simulink model "Control_LIM_H9"  (R2025b)
settings: Solver=VariableStepAuto  StartTime=0.0  StopTime=10  RelTol=1e-3
undefined symbols (not defined in the file): a, airgap, b, corriente, dent_lsm, force_lsm, frecuencia_acel, frecuencia_freno, fuerza, fuerza_drag, FuerzaX_freno, kd, magnitude, masa_pod, paso_polar, r, slip, vel_motor_freno, velocidad_drag
libraries: slpidlib x3, eeTransforms x1
(part 1 of 2)
settings Model: NumberOfSteps=1500000  Creator=Siulesoj5  LastModifiedBy=Lenovo
settings RTWCC: GPUComputeCapability=3.5

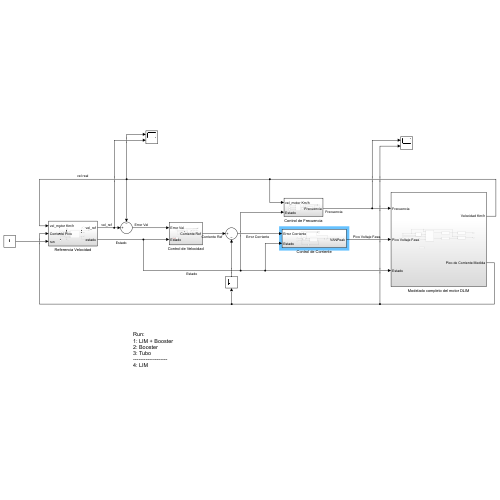
[thumbnail: Simulink's stored preview of the top-level diagram]
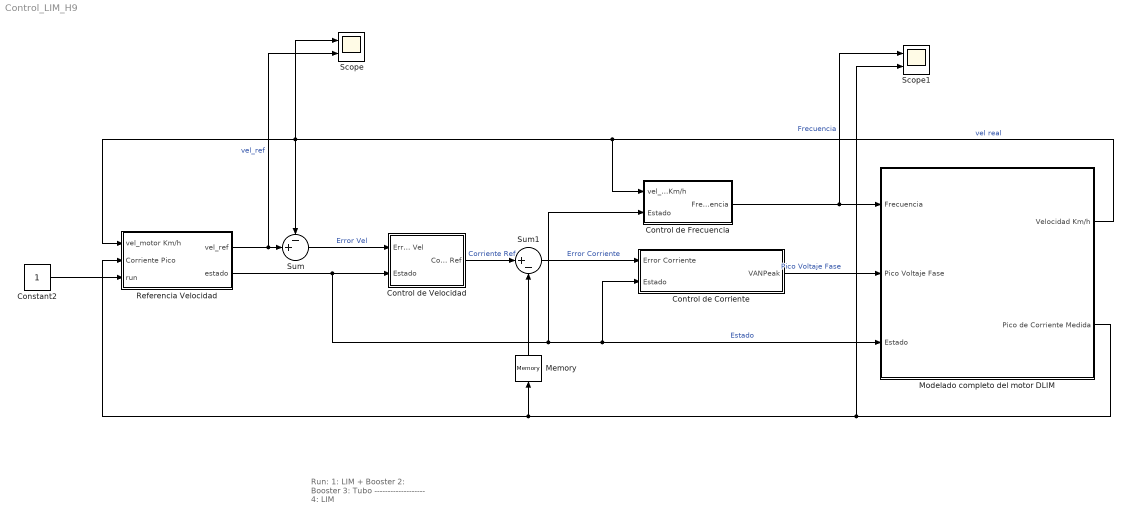
== system Control_LIM_H9 ==
  note: Run:
      | 1: LIM + Booster
      | 2: Booster
      | 3: Tubo
      | -------------------
      | 4: LIM
  Constant2 : Constant  OutMin=1  OutMax=4  OutDataTypeStr=int16
  Control de Corriente : Subsystem
  Control de Frecuencia : Subsystem
  Control de Velocidad : Subsystem
  Memory : Memory
  Modelado completo del motor DLIM : Subsystem
  Referencia Velocidad : Subsystem
  Scope : Scope  NumInputPorts=2
      settings: ActiveDisplayYMinimum=-1  ActiveDisplayYMaximum=1  DataLoggingVariableName=ScopeData19
  Scope1 : Scope  NumInputPorts=2
      settings: ActiveDisplayYMinimum=-1  ActiveDisplayYMaximum=1  DataLoggingVariableName=ScopeData20
  Sum : Sum  Inputs=-+|
  Sum1 : Sum  Inputs=|+-
  wires:
  Referencia Velocidad/1(vel_ref) -> Scope/2, Sum/2  "vel_ref"
  Sum/1 -> Control de Velocidad/1(Error Vel)  "Error Vel"
  Control de Velocidad/1(Corriente Ref) -> Sum1/1  "Corriente Ref"
  Sum1/1 -> Control de Corriente/1(Error Corriente)  "Error Corriente"
  Referencia Velocidad/2(estado) -> Modelado completo del motor DLIM/3(Estado), Control de Corriente/2(Estado), Control de Frecuencia/2(Estado), Control de Velocidad/2(Estado)  "Estado"
  Memory/1 -> Sum1/2
  Constant2/1 -> Referencia Velocidad/3(run)
  Modelado completo del motor DLIM/2(Pico de Corriente Medida) -> Referencia Velocidad/2(Corriente Pico), Memory/1, Scope1/2
  Modelado completo del motor DLIM/1(Velocidad Km/h) -> Scope/1, Sum/1, Referencia Velocidad/1(vel_motor Km/h), Control de Frecuencia/1(vel_motor Km/h)  "vel real"
  Control de Frecuencia/1(Frecuencia) -> Scope1/1, Modelado completo del motor DLIM/1(Frecuencia)  "Frecuencia"
  Control de Corriente/1(VANPeak) -> Modelado completo del motor DLIM/2(Pico Voltaje Fase)  "Pico Voltaje Fase"

== system Control_LIM_H9/Control de Corriente ==
  Error Corriente : Inport
  Estado : Inport  Port=2
  MATLAB Function : MATLAB Function  TreatAsAtomicUnit=on
  Memory : Memory
  PID Controller : slpidlib/PID Controller  Controller=PI  Form=Parallel  TimeDomain=Discrete-time  UseExternalTs=off  SampleTime=0.0002  IntegratorMethod=Forward Euler  FilterMethod=Forward Euler  ControllerParametersSource=internal  P=1  I=12  UseKiTs=off  D=0  UseExternalDerivativeSource=off  N=100  UseFilter=on  TunerSelectOption=Transfer Function Based (PID Tuner App)  InitialConditionSource=internal  InitialConditionForIntegrator=0  InitialConditionForFilter=0  DifferentiatorICPrevScaledInput=0  ExternalReset=level  TrackingMode=off  Kt=1  LimitOutput=off  SatLimitsSource=internal  UpperSaturationLimit=inf  LowerSaturationLimit=-inf  LinearizeAsGain=on  AntiWindupMode=none  Kb=1  LimitIntegrator=off  UpperIntegratorSaturationLimit=inf  LowerIntegratorSaturationLimit=-inf  POutMin=[]  POutMax=[]  IOutMin=[]  IOutMax=[]  DOutMin=[]  DOutMax=[]  NOutMin=[]  NOutMax=[]  SumOutMin=[]  SumOutMax=[]  SaturationOutMin=[]  SaturationOutMax=[]  PParamMin=[]  PParamMax=[]  IParamMin=[]  IParamMax=[]  DParamMin=[]  DParamMax=[]  NParamMin=[]  NParamMax=[]  KbParamMin=[]  KbParamMax=[]  KtParamMin=[]  KtParamMax=[]  KbOutMin=[]  KbOutMax=[]  KtOutMin=[]  KtOutMax=[]  IntegratorOutMin=[]  IntegratorOutMax=[]  FilterOutMin=[]  FilterOutMax=[]  SumI1OutMin=[]  SumI1OutMax=[]  SumI2OutMin=[]  SumI2OutMax=[]  SumI3OutMin=[]  SumI3OutMax=[]  SumI4OutMin=[]  SumI4OutMax=[]  SumDOutMin=[]  SumDOutMax=[]  DifferentiatorOutMin=[]  DifferentiatorOutMax=[]  FilterDiffOutCoefMin=[]  FilterDiffOutCoefMax=[]  ReciprocalOutMin=[]  ReciprocalOutMax=[]  SumDenOutMin=[]  SumDenOutMax=[]  SumNumOutMin=[]  SumNumOutMax=[]  DivideOutMin=[]  DivideOutMax=[]  UdiffTsProdOutMin=[]  UdiffTsProdOutMax=[]  NTsProdOutMin=[]  NTsProdOutMax=[]  UintegralTsProdOutMin=[]  UintegralTsProdOutMax=[]  UngainTsProdOutMin=[]  UngainTsProdOutMax=[]  ClampingZeroOutDataTypeStr=Inherit: Inherit via back propagation  ClampingZeroOutMin=[]  ClampingZeroOutMax=[]  FilterDenConstantOutDataTypeStr=Inherit: Inherit via back propagation  FilterDenConstantOutMin=[]  FilterDenConstantOutMax=[]  PCopyOutDataTypeStr=Inherit: Inherit via back propagation  PCopyOutMin=[]  PCopyOutMax=[]  NCopyOutDataTypeStr=Inherit: Inherit via back propagation  NCopyOutMin=[]  NCopyOutMax=[]  IntegratorContinuousStateAttributes=''  IntegratorStateMustResolveToSignalObject=off  IntegratorRTWStateStorageClass=Auto  FilterContinuousStateAttributes=''  FilterStateMustResolveToSignalObject=off  FilterRTWStateStorageClass=Auto  ParallelPVariant=InternalParameters  IdealPVariant=Disabled  IVariant=InternalParameters  DVariant=Disabled  IntegratorVariant=Discrete  SatVariant=Disabled  AWVariant=Passthrough  PCopyVariant=Disabled  TRVariant=Disabled  FdbkBlocksVariant=Forward  IdealPFdbkVariant=Disabled  SatFdbkVariant=Disabled  DerivativeFilterVariant=Disabled  NVariant=Disabled  NCopyVariant=Disabled_SignalSpec  FilterICVariant=Disabled  IntegratorICVariant=InternalICs  ExternalResetVariant=ExternalReset  TRSumVariant=Passthrough  SumFdbkVariant=Disabled  SumVariant=Sum_PI  TsampFilterVariant=InternalTs  TsampNgainVariant=Passthrough  TsampIntegralVariant=Disabled_SignalSpec  ExternalSaturationOutDataTypeStr=Inherit: Same as second input  DerivativeSourceVariant=Disabled  PreIntVariant=InternalPreInt
  Saturation : Saturate  UpperLimit=250*(sqrt(3)/2)/sqrt(3)  LowerLimit=0
  Scope : Scope  NumInputPorts=3
      settings: ActiveDisplayYMinimum=-76.56634  ActiveDisplayYMaximum=118.49234  DataLoggingVariableName=ScopeData5
  VANPeak : Outport
  wires:
  Error Corriente/1 -> Scope/1, PID Controller/1
  PID Controller/1 -> Scope/2, MATLAB Function/1(corriente)
  Saturation/1 -> Scope/3, VANPeak/1
  MATLAB Function/1(pico_voltaje) -> Saturation/1
  Estado/1 -> MATLAB Function/2(estado)
  MATLAB Function/2(reset) -> Memory/1
  Memory/1 -> PID Controller/2

== system Control_LIM_H9/Control de Frecuencia ==
  vel_motor Km/h : Inport
  Estado : Inport  Port=2
  Constant : Constant  Value=a
  Constant1 : Constant  Value=b
  Constant2 : Constant  Value=-3
  MATLAB Function : MATLAB Function  TreatAsAtomicUnit=on
  MATLAB Function1 : MATLAB Function  TreatAsAtomicUnit=on
  Scope : Scope  NumInputPorts=3
      settings: ActiveDisplayYMinimum=29.835238215543111  ActiveDisplayYMaximum=30.084237893487973
  Frecuencia : Outport
  wires:
  vel_motor Km/h/1 -> MATLAB Function/1(vel)
  MATLAB Function/1(frecuencia) -> Scope/1, MATLAB Function1/1(f_acel)  "f_aceleracion"
  MATLAB Function1/1(f) -> Scope/3, Frecuencia/1  "f_actual"
  Constant/1 -> MATLAB Function/2(a)
  Constant1/1 -> MATLAB Function/3(b)
  Constant2/1 -> Scope/2, MATLAB Function1/2(f_frenado)  "f_frenado"
  Estado/1 -> MATLAB Function1/3(estado)

== system Control_LIM_H9/Control de Velocidad ==
  Error Vel : Inport
  Estado : Inport  Port=2
  Abs : Abs  ZeroCross=off  SaturateOnIntegerOverflow=off
  Abs1 : Abs  SaturateOnIntegerOverflow=off
  MATLAB Function : MATLAB Function  TreatAsAtomicUnit=on
  MATLAB Function1 : MATLAB Function  TreatAsAtomicUnit=on
  Memory : Memory
  PID Controller : slpidlib/PID Controller  Controller=PI  Form=Parallel  TimeDomain=Discrete-time  UseExternalTs=off  SampleTime=0.001  IntegratorMethod=Forward Euler  FilterMethod=Forward Euler  ControllerParametersSource=internal  P=9  I=1  UseKiTs=off  D=0  UseExternalDerivativeSource=off  N=100  UseFilter=on  TunerSelectOption=Transfer Function Based (PID Tuner App)  InitialConditionSource=internal  InitialConditionForIntegrator=0  InitialConditionForFilter=0  DifferentiatorICPrevScaledInput=0  ExternalReset=level  TrackingMode=off  Kt=1  LimitOutput=off  SatLimitsSource=internal  UpperSaturationLimit=inf  LowerSaturationLimit=-inf  LinearizeAsGain=on  AntiWindupMode=none  Kb=1  LimitIntegrator=off  UpperIntegratorSaturationLimit=inf  LowerIntegratorSaturationLimit=-inf  POutMin=[]  POutMax=[]  IOutMin=[]  IOutMax=[]  DOutMin=[]  DOutMax=[]  NOutMin=[]  NOutMax=[]  SumOutMin=[]  SumOutMax=[]  SaturationOutMin=[]  SaturationOutMax=[]  PParamMin=[]  PParamMax=[]  IParamMin=[]  IParamMax=[]  DParamMin=[]  DParamMax=[]  NParamMin=[]  NParamMax=[]  KbParamMin=[]  KbParamMax=[]  KtParamMin=[]  KtParamMax=[]  KbOutMin=[]  KbOutMax=[]  KtOutMin=[]  KtOutMax=[]  IntegratorOutMin=[]  IntegratorOutMax=[]  FilterOutMin=[]  FilterOutMax=[]  SumI1OutMin=[]  SumI1OutMax=[]  SumI2OutMin=[]  SumI2OutMax=[]  SumI3OutMin=[]  SumI3OutMax=[]  SumI4OutMin=[]  SumI4OutMax=[]  SumDOutMin=[]  SumDOutMax=[]  DifferentiatorOutMin=[]  DifferentiatorOutMax=[]  FilterDiffOutCoefMin=[]  FilterDiffOutCoefMax=[]  ReciprocalOutMin=[]  ReciprocalOutMax=[]  SumDenOutMin=[]  SumDenOutMax=[]  SumNumOutMin=[]  SumNumOutMax=[]  DivideOutMin=[]  DivideOutMax=[]  UdiffTsProdOutMin=[]  UdiffTsProdOutMax=[]  NTsProdOutMin=[]  NTsProdOutMax=[]  UintegralTsProdOutMin=[]  UintegralTsProdOutMax=[]  UngainTsProdOutMin=[]  UngainTsProdOutMax=[]  ClampingZeroOutDataTypeStr=Inherit: Inherit via back propagation  ClampingZeroOutMin=[]  ClampingZeroOutMax=[]  FilterDenConstantOutDataTypeStr=Inherit: Inherit via back propagation  FilterDenConstantOutMin=[]  FilterDenConstantOutMax=[]  PCopyOutDataTypeStr=Inherit: Inherit via back propagation  PCopyOutMin=[]  PCopyOutMax=[]  NCopyOutDataTypeStr=Inherit: Inherit via back propagation  NCopyOutMin=[]  NCopyOutMax=[]  IntegratorContinuousStateAttributes=''  IntegratorStateMustResolveToSignalObject=off  IntegratorRTWStateStorageClass=Auto  FilterContinuousStateAttributes=''  FilterStateMustResolveToSignalObject=off  FilterRTWStateStorageClass=Auto  ParallelPVariant=InternalParameters  IdealPVariant=Disabled  IVariant=InternalParameters  DVariant=Disabled  IntegratorVariant=Discrete  SatVariant=Disabled  AWVariant=Passthrough  PCopyVariant=Disabled  TRVariant=Disabled  FdbkBlocksVariant=Forward  IdealPFdbkVariant=Disabled  SatFdbkVariant=Disabled  DerivativeFilterVariant=Disabled  NVariant=Disabled  NCopyVariant=Disabled_SignalSpec  FilterICVariant=Disabled  IntegratorICVariant=InternalICs  ExternalResetVariant=ExternalReset  TRSumVariant=Passthrough  SumFdbkVariant=Disabled  SumVariant=Sum_PI  TsampFilterVariant=InternalTs  TsampNgainVariant=Passthrough  TsampIntegralVariant=Disabled_SignalSpec  ExternalSaturationOutDataTypeStr=Inherit: Same as second input  DerivativeSourceVariant=Disabled  PreIntVariant=InternalPreInt
  PID Controller1 : slpidlib/PID Controller  Controller=PI  Form=Parallel  TimeDomain=Continuous-time  UseExternalTs=off  SampleTime=-1  IntegratorMethod=Forward Euler  FilterMethod=Forward Euler  ControllerParametersSource=internal  P=1  I=1  UseKiTs=off  D=0  UseExternalDerivativeSource=off  N=100  UseFilter=on  TunerSelectOption=Transfer Function Based (PID Tuner App)  InitialConditionSource=internal  InitialConditionForIntegrator=0  InitialConditionForFilter=0  DifferentiatorICPrevScaledInput=0  ExternalReset=none  TrackingMode=off  Kt=1  LimitOutput=off  SatLimitsSource=internal  UpperSaturationLimit=inf  LowerSaturationLimit=-inf  LinearizeAsGain=on  AntiWindupMode=none  Kb=1  LimitIntegrator=off  UpperIntegratorSaturationLimit=inf  LowerIntegratorSaturationLimit=-inf  POutMin=[]  POutMax=[]  IOutMin=[]  IOutMax=[]  DOutMin=[]  DOutMax=[]  NOutMin=[]  NOutMax=[]  SumOutMin=[]  SumOutMax=[]  SaturationOutMin=[]  SaturationOutMax=[]  PParamMin=[]  PParamMax=[]  IParamMin=[]  IParamMax=[]  DParamMin=[]  DParamMax=[]  NParamMin=[]  NParamMax=[]  KbParamMin=[]  KbParamMax=[]  KtParamMin=[]  KtParamMax=[]  KbOutMin=[]  KbOutMax=[]  KtOutMin=[]  KtOutMax=[]  IntegratorOutMin=[]  IntegratorOutMax=[]  FilterOutMin=[]  FilterOutMax=[]  SumI1OutMin=[]  SumI1OutMax=[]  SumI2OutMin=[]  SumI2OutMax=[]  SumI3OutMin=[]  SumI3OutMax=[]  SumI4OutMin=[]  SumI4OutMax=[]  SumDOutMin=[]  SumDOutMax=[]  DifferentiatorOutMin=[]  DifferentiatorOutMax=[]  FilterDiffOutCoefMin=[]  FilterDiffOutCoefMax=[]  ReciprocalOutMin=[]  ReciprocalOutMax=[]  SumDenOutMin=[]  SumDenOutMax=[]  SumNumOutMin=[]  SumNumOutMax=[]  DivideOutMin=[]  DivideOutMax=[]  UdiffTsProdOutMin=[]  UdiffTsProdOutMax=[]  NTsProdOutMin=[]  NTsProdOutMax=[]  UintegralTsProdOutMin=[]  UintegralTsProdOutMax=[]  UngainTsProdOutMin=[]  UngainTsProdOutMax=[]  ClampingZeroOutDataTypeStr=Inherit: Inherit via back propagation  ClampingZeroOutMin=[]  ClampingZeroOutMax=[]  FilterDenConstantOutDataTypeStr=Inherit: Inherit via back propagation  FilterDenConstantOutMin=[]  FilterDenConstantOutMax=[]  PCopyOutDataTypeStr=Inherit: Inherit via back propagation  PCopyOutMin=[]  PCopyOutMax=[]  NCopyOutDataTypeStr=Inherit: Inherit via back propagation  NCopyOutMin=[]  NCopyOutMax=[]  IntegratorContinuousStateAttributes=''  IntegratorStateMustResolveToSignalObject=off  IntegratorRTWStateStorageClass=Auto  FilterContinuousStateAttributes=''  FilterStateMustResolveToSignalObject=off  FilterRTWStateStorageClass=Auto  ParallelPVariant=InternalParameters  IdealPVariant=Disabled  IVariant=InternalParameters  DVariant=Disabled  IntegratorVariant=Continuous  SatVariant=Disabled  AWVariant=Passthrough  PCopyVariant=Disabled  TRVariant=Disabled  FdbkBlocksVariant=Forward  IdealPFdbkVariant=Disabled  SatFdbkVariant=Disabled  DerivativeFilterVariant=Disabled  NVariant=Disabled  NCopyVariant=Disabled_SignalSpec  FilterICVariant=Disabled  IntegratorICVariant=InternalICs  ExternalResetVariant=Disabled  TRSumVariant=Passthrough  SumFdbkVariant=Disabled  SumVariant=Sum_PI  TsampFilterVariant=InternalTs  TsampNgainVariant=Passthrough  TsampIntegralVariant=Disabled_SignalSpec  ExternalSaturationOutDataTypeStr=Inherit: Same as second input  DerivativeSourceVariant=Disabled  PreIntVariant=InternalPreInt
  Saturation : Saturate  UpperLimit=100  LowerLimit=-100
  Scope : Scope  NumInputPorts=5
      settings: ActiveDisplayYMinimum=-64.17635  ActiveDisplayYMaximum=47.1097  DataLoggingVariableName=ScopeData4
  Scope1 : Scope
      settings: ActiveDisplayYMinimum=-0.875  ActiveDisplayYMaximum=7.875  DataLoggingVariableName=ScopeData5
  Scope2 : Scope  NumInputPorts=2
      settings: ActiveDisplayYMinimum=-56.2709708249014  ActiveDisplayYMaximum=506.43873742411267  DataLoggingVariableName=ScopeData24
  Corriente Ref : Outport
  wires:
  Estado/1 -> Scope1/1, MATLAB Function/2(estado)
  MATLAB Function/1(i_ref) -> Scope2/2, Saturation/1  "i_ref sin saturar"
  Abs/1 -> Corriente Ref/1, Scope/5
  MATLAB Function/2(reset) -> Memory/1
  Memory/1 -> PID Controller/2
  Saturation/1 -> Scope2/1, Abs/1, Scope/4  "i_ref saturada"
  PID Controller/1 -> Scope/3, MATLAB Function/1(i)
  ? -> MATLAB Function1/2(normal)
  Abs1/1 -> MATLAB Function1/1(abs)
  ? -> MATLAB Function1/3(estado)
  ? -> Abs1/1
  Error Vel/1 -> Scope/1, Scope/2, PID Controller/1

== system Control_LIM_H9/Modelado completo del motor DLIM ==
  Frecuencia : Inport
  Pico Voltaje Fase : Inport  Port=2
  Estado : Inport  Port=3
  Constant1 : Constant  OutMin=1  OutMax=4  OutDataTypeStr=double
  Cálculo Máximo : Subsystem
  Cálculo Velocidad : Subsystem
  Integración Booster : Subsystem  Commented=on
  Inversor Trifásico : Subsystem
  LIM Model : Subsystem
  Sensor IMU : Subsystem
  Sensor de Corriente : Subsystem
  Velocidad Km/h : Outport
  Pico de Corriente Medida : Outport  Port=2
  wires:
  Sensor IMU/1(Acel_IMU) -> Cálculo Velocidad/1(acel m/s^2)  "Aceleración m/s^2"
  LIM Model/2(Corriente UVW) -> Sensor de Corriente/1(Corriente UVW)  "Corriente Real"
  Inversor Trifásico/1(VFaseN) -> LIM Model/2(VFaseN)
  Pico Voltaje Fase/1 -> Inversor Trifásico/2(VUNPeak)
  Constant1/1 -> LIM Model/4(Fuerza_lsm)
  Sensor de Corriente/1(Corriente Medida) -> Cálculo Máximo/2(Corriente Medida)  "Corriente Medida"
  Frecuencia/1 -> LIM Model/1(Frecuencia), Cálculo Máximo/1(Frecuencia), Inversor Trifásico/1(Frecuencia)
  LIM Model/1(Acel (m/s^2)) -> Sensor IMU/1(Acel)  "Aceleración Real"
  Cálculo Máximo/1(Corriente Pico) -> Pico de Corriente Medida/1  "Pico de Corriente Medida"
  Estado/1 -> LIM Model/3(Estado)
  Cálculo Velocidad/1(vel_motor Km/h) -> Velocidad Km/h/1  "Velocidad Km/h"

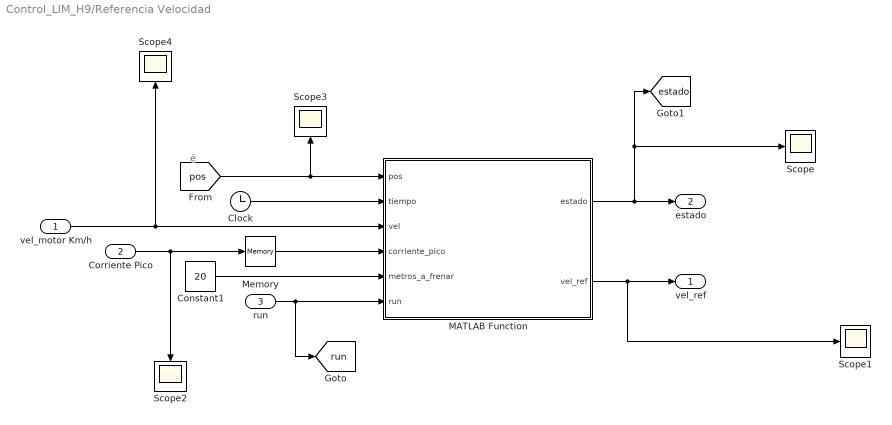
== system Control_LIM_H9/Referencia Velocidad ==
  note: é
  vel_motor Km/h : Inport
  Corriente Pico : Inport  Port=2
  run : Inport  Port=3
  Clock : Clock
  Constant1 : Constant  Value=20
  MATLAB Function : MATLAB Function  TreatAsAtomicUnit=on
  Memory : Memory
  Scope{,1..4} (5 alike) : Scope
      Scope settings: ActiveDisplayYMinimum=-0.875  ActiveDisplayYMaximum=7.875  DataLoggingVariableName=ScopeData2
      Scope1 settings: ActiveDisplayYMinimum=-6.25  ActiveDisplayYMaximum=56.25  DataLoggingVariableName=ScopeData3
      Scope2 settings: ActiveDisplayYMinimum=-11.77656  ActiveDisplayYMaximum=109.65201  DataLoggingVariableName=ScopeData11
      Scope3 settings: ActiveDisplayYMinimum=-4.42643  ActiveDisplayYMaximum=39.83783  DataLoggingVariableName=ScopeData12
      Scope4 settings: ActiveDisplayYMinimum=-6.27724  ActiveDisplayYMaximum=56.25913  DataLoggingVariableName=ScopeData4
  vel_ref : Outport
  estado : Outport  Port=2
  tag scope: estado=global, run=global
  wires:
  MATLAB Function/1(estado) -> [estado], Scope/1, estado/1
  Corriente Pico/1 -> Memory/1, Scope2/1
  Memory/1 -> MATLAB Function/4(corriente_pico)
  Constant1/1 -> MATLAB Function/5(metros_a_frenar)
  vel_motor Km/h/1 -> Scope4/1, MATLAB Function/3(vel)
  MATLAB Function/2(vel_ref) -> vel_ref/1, Scope1/1
  Clock/1 -> MATLAB Function/2(tiempo)
  [pos] -> MATLAB Function/1(pos), Scope3/1
  run/1 -> MATLAB Function/6(run), [run]

== system Control_LIM_H9/Modelado completo del motor DLIM/Cálculo Máximo ==
  Frecuencia : Inport
  Corriente Medida : Inport  Port=2
  Clock : Clock
  MATLAB Function : MATLAB Function  TreatAsAtomicUnit=on
  Scope : Scope  NumInputPorts=2
      settings: ActiveDisplayYMinimum=-131.22711  ActiveDisplayYMaximum=131.22711  DataLoggingVariableName=ScopeData3
  Corriente Pico : Outport
  wires:
  Frecuencia/1 -> MATLAB Function/1(frecuencia)
  MATLAB Function/1(maximo) -> Scope/1, Corriente Pico/1
  Corriente Medida/1 -> Scope/2, MATLAB Function/2(valores)
  Clock/1 -> MATLAB Function/3(tiempo)

== system Control_LIM_H9/Modelado completo del motor DLIM/Cálculo Velocidad ==
  acel m/s^2 : Inport
  Gain : Gain  Gain=3.6
  Integrator : Integrator
  Integrator1 : Integrator  InitialCondition=3/3.6
  MATLAB Function : MATLAB Function  TreatAsAtomicUnit=on
  Scope : Scope
      settings: ActiveDisplayYMinimum=-6.21369  ActiveDisplayYMaximum=55.85682
  Scope1 : Scope
      settings: ActiveDisplayYMinimum=-1  ActiveDisplayYMaximum=1  DataLoggingVariableName=ScopeData2
  Scope2 : Scope
      settings: ActiveDisplayYMinimum=-1  ActiveDisplayYMaximum=1  DataLoggingVariableName=ScopeData3
  vel_motor Km/h : Outport
  wires:
  MATLAB Function/1(vel) -> Gain/1  "vel_motor m/s"
  Gain/1 -> Scope/1, vel_motor Km/h/1  "vel_motor Km/h"
  acel m/s^2/1 -> Scope2/1, Integrator1/1, Integrator/1
  [run] -> MATLAB Function/3(run)
  Integrator1/1 -> MATLAB Function/2(vel2)  "vel_motor m/s"
  Integrator/1 -> Scope1/1, MATLAB Function/1(vel1)  "vel_motor m/s"

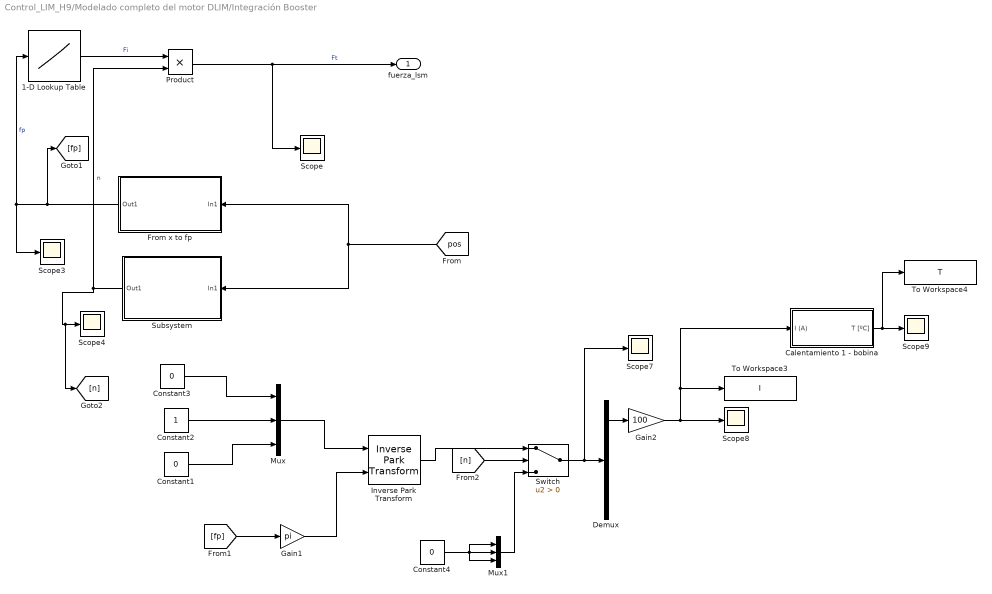
== system Control_LIM_H9/Modelado completo del motor DLIM/Integración Booster ==
  1-D Lookup Table : Lookup_n-D  NumberOfTableDimensions=1  BreakpointsForDimension1=dent_lsm  Table=force_lsm  InternalRulePriority=Speed  RndMeth=Simplest
  Calentamiento 1 - bobina : Subsystem
  Constant1 : Constant  Value=0
  Constant2 : Constant
  Constant3 : Constant  Value=0
  Constant4 : Constant  Value=0
  Demux : Demux  Outputs=3
  From x to fp : Subsystem
  Gain1 : Gain  Gain=pi
  Gain2 : Gain  Gain=100
  Inverse Park Transform : eeTransforms/Inverse Park Transform  AxisAlignment=Q-axis  PowerInvariant=off
      settings: LibrarySourceBlock=|
      | ee_sl_lib/Mathematical
      | Transforms/Inverse
      | Park Transform
  Mux : Mux  Inputs=3
  Mux1 : Mux  Inputs=3
  Product : Product
  Scope{,3..4,7..9} (6 alike) : Scope
      Scope settings: ActiveDisplayYMinimum=-398.29312  ActiveDisplayYMaximum=3584.6381  DataLoggingVariableName=ScopeData12
      Scope3 settings: ActiveDisplayYMinimum=-0.25  ActiveDisplayYMaximum=2.25  DataLoggingVariableName=ScopeData4
      Scope4 settings: ActiveDisplayYMinimum=-0.75  ActiveDisplayYMaximum=6.75  DataLoggingVariableName=ScopeData5
      Scope7 settings: ActiveDisplayYMinimum=-1.25  ActiveDisplayYMaximum=1.25  DataLoggingVariableName=ScopeData8
      Scope8 settings: ActiveDisplayYMinimum=-124.99997  ActiveDisplayYMaximum=125  DataLoggingVariableName=ScopeData9
      Scope9 settings: ActiveDisplayYMinimum=54.98266  ActiveDisplayYMaximum=57.13779  DataLoggingVariableName=ScopeData10
  Subsystem : Subsystem
  Switch : Switch  Criteria=u2 > Threshold  SaturateOnIntegerOverflow=off  InputSameDT=off
  To Workspace3 : ToWorkspace  VariableName=I  SaveFormat=Timeseries  SampleTime=-1
  To Workspace4 : ToWorkspace  VariableName=T  SaveFormat=Timeseries  SampleTime=-1
  fuerza_lsm : Outport
  wires:
  [n] -> Switch/2
  Subsystem/1(Out1) -> Product/2, [n], Scope4/1  "n"
  [fp] -> Gain1/1
  Constant2/1 -> Mux/2
  Mux/1 -> Inverse Park Transform/1
  Inverse Park Transform/1 -> Switch/1
  Demux/1 -> Gain2/1
  Constant1/1 -> Mux/3
  Constant3/1 -> Mux/1
  1-D Lookup Table/1 -> Product/1  "Fi"
  Constant4/1 -> Mux1/3, Mux1/1, Mux1/2
  Gain1/1 -> Inverse Park Transform/2
  From x to fp/1(Out1) -> [fp], 1-D Lookup Table/1, Scope3/1  "fp"
  Product/1 -> Scope/1, fuerza_lsm/1  "Ft"
  Mux1/1 -> Switch/3
  Gain2/1 -> Calentamiento 1 - bobina/1(I (A)), To Workspace3/1, Scope8/1
  Switch/1 -> Scope7/1, Demux/1
  Calentamiento 1 - bobina/1(T [ºC]) -> To Workspace4/1, Scope9/1
  [pos] -> From x to fp/1(In1), Subsystem/1(In1)

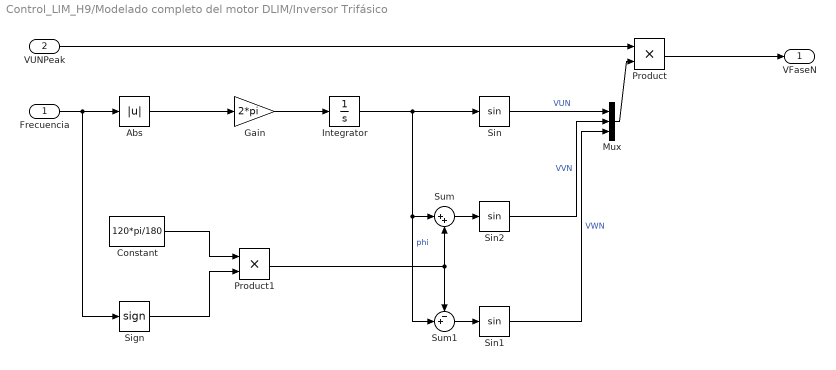
== system Control_LIM_H9/Modelado completo del motor DLIM/Inversor Trifásico ==
  Frecuencia : Inport
  VUNPeak : Inport  Port=2
  Abs : Abs  SaturateOnIntegerOverflow=off
  Constant : Constant  Value=120*pi/180
  Gain : Gain  Gain=2*pi
  Integrator : Integrator  WrapState=on  WrappedStateUpperValue=2*pi  WrappedStateLowerValue=0
  Mux : Mux  Inputs=3
  Product : Product
  Product1 : Product
  Sign : Signum
  Sin : Trigonometry
  Sin1 : Trigonometry
  Sin2 : Trigonometry
  Sum : Sum  Inputs=|++
  Sum1 : Sum  Inputs=-+|
  VFaseN : Outport
  wires:
  VUNPeak/1 -> Product/1
  Frecuencia/1 -> Abs/1, Sign/1
  Gain/1 -> Integrator/1
  Integrator/1 -> Sin/1, Sum/1, Sum1/2  "phi"
  Product/1 -> VFaseN/1
  Mux/1 -> Product/2
  Sin/1 -> Mux/1  "VUN"
  Abs/1 -> Gain/1
  Constant/1 -> Product1/1
  Sign/1 -> Product1/2
  Sin2/1 -> Mux/2  "VVN"
  Sin1/1 -> Mux/3  "VWN"
  Sum/1 -> Sin2/1
  Sum1/1 -> Sin1/1
  Product1/1 -> Sum/2, Sum1/1

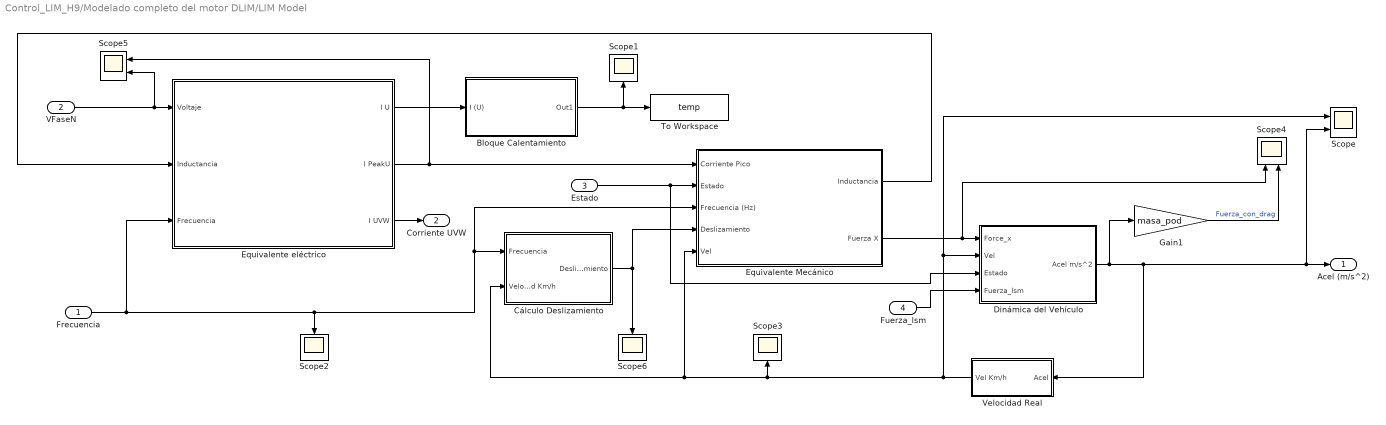
== system Control_LIM_H9/Modelado completo del motor DLIM/LIM Model ==
  Frecuencia : Inport
  VFaseN : Inport  Port=2
  Estado : Inport  Port=3
  Fuerza_lsm : Inport  Port=4  OutDataTypeStr=double
  Bloque Calentamiento : Subsystem
  Cálculo Deslizamiento : Subsystem
  Dinámica del Vehículo : Subsystem
  Equivalente Mecánico : Subsystem
  Equivalente eléctrico : Subsystem
  Gain1 : Gain  Gain=masa_pod
  Scope : Scope  NumInputPorts=2
      settings: ActiveDisplayYMinimum=-3.92278  ActiveDisplayYMaximum=27.40382  DataLoggingVariableName=ScopeData8
  Scope{1..3,6} (4 alike) : Scope
      Scope1 settings: ActiveDisplayYMinimum=38.64676  ActiveDisplayYMaximum=52.17914  DataLoggingVariableName=ScopeData14
      Scope2 settings: ActiveDisplayYMinimum=-8.38399  ActiveDisplayYMaximum=45.45589  DataLoggingVariableName=ScopeData15
      Scope3 settings: ActiveDisplayYMinimum=-6.37396  ActiveDisplayYMaximum=56.13927  DataLoggingVariableName=ScopeData17
      Scope6 settings: ActiveDisplayYMinimum=0.18342  ActiveDisplayYMaximum=0.26007  DataLoggingVariableName=ScopeData2
  Scope4 : Scope  NumInputPorts=2
      settings: ActiveDisplayYMinimum=-3197.10716  ActiveDisplayYMaximum=1490.72148  DataLoggingVariableName=ScopeData18
  Scope5 : Scope  NumInputPorts=2
      settings: ActiveDisplayYMinimum=-156.25  ActiveDisplayYMaximum=156.25
  To Workspace : ToWorkspace  VariableName=temp  SaveFormat=Timeseries  SampleTime=-1
  Velocidad Real : Subsystem
  Acel (m/s^2) : Outport
  Corriente UVW : Outport  Port=2
  wires:
  VFaseN/1 -> Equivalente eléctrico/1(Voltaje), Scope5/2
  Equivalente eléctrico/3(I UVW) -> Corriente UVW/1
  Estado/1 -> Dinámica del Vehículo/3(Estado), Equivalente Mecánico/2(Estado)
  Equivalente eléctrico/2(I PeakU) -> Scope5/1, Equivalente Mecánico/1(Corriente Pico)
  Dinámica del Vehículo/1(Acel m/s^2) -> Gain1/1, Scope/2, Acel (m/s^2)/1, Velocidad Real/1(Acel)
  Velocidad Real/1(Vel Km/h) -> Scope/1, Dinámica del Vehículo/2(Vel), Cálculo Deslizamiento/2(Velocidad Km/h), Equivalente Mecánico/5(Vel), Scope3/1
  Cálculo Deslizamiento/1(Deslizamiento) -> Equivalente Mecánico/4(Deslizamiento), Scope6/1
  Equivalente Mecánico/1(Inductancia) -> Equivalente eléctrico/2(Inductancia)
  Equivalente eléctrico/1(I U) -> Bloque Calentamiento/1(I (U))
  Bloque Calentamiento/1(Out1) -> To Workspace/1, Scope1/1
  Frecuencia/1 -> Equivalente eléctrico/3(Frecuencia), Scope2/1, Equivalente Mecánico/3(Frecuencia (Hz)), Cálculo Deslizamiento/1(Frecuencia)
  Equivalente Mecánico/2(Fuerza X) -> Scope4/1, Dinámica del Vehículo/1(Force_x)
  Fuerza_lsm/1 -> Dinámica del Vehículo/4(Fuerza_lsm)
  Gain1/1 -> Scope4/2  "Fuerza_con_drag"

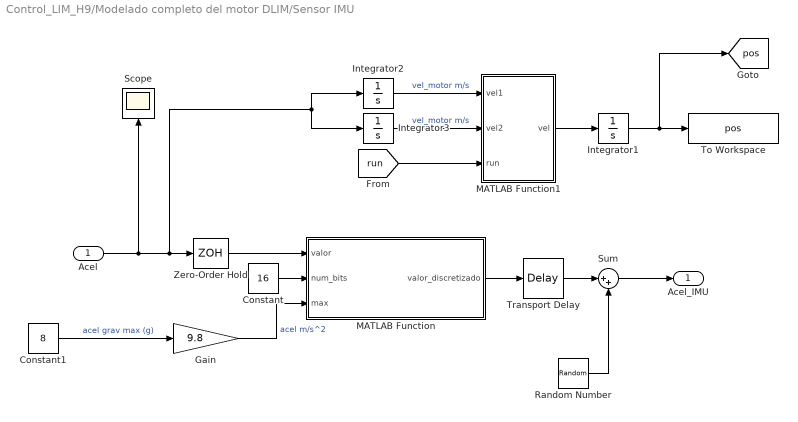
== system Control_LIM_H9/Modelado completo del motor DLIM/Sensor IMU ==
  Acel : Inport
  Constant : Constant  Value=16
  Constant1 : Constant  Value=8
  Gain : Gain  Gain=9.8
  Integrator1 : Integrator
  Integrator2 : Integrator
  Integrator3 : Integrator  InitialCondition=3/3.6
  MATLAB Function : MATLAB Function  TreatAsAtomicUnit=on
  MATLAB Function1 : MATLAB Function  TreatAsAtomicUnit=on
  Random Number : RandomNumber  Variance=0.1  SampleTime=0.001
  Scope : Scope
      settings: ActiveDisplayYMinimum=-0.65188  ActiveDisplayYMaximum=5.54198  DataLoggingVariableName=ScopeData13
  Sum : Sum  Inputs=|++
  To Workspace : ToWorkspace  VariableName=pos  SaveFormat=Timeseries  SampleTime=-1
  Transport Delay : TransportDelay  DelayTime=0.001
  Zero-Order Hold : ZeroOrderHold  SampleTime=0.001
  Acel_IMU : Outport
  tag scope: pos=global
  wires:
  MATLAB Function/1(valor_discretizado) -> Transport Delay/1
  Constant/1 -> MATLAB Function/2(num_bits)
  Constant1/1 -> Gain/1  "acel grav max (g)"
  Gain/1 -> MATLAB Function/3(max)  "acel m/s^2"
  MATLAB Function1/1(vel) -> Integrator1/1
  Sum/1 -> Acel_IMU/1
  Integrator1/1 -> [pos], To Workspace/1
  Random Number/1 -> Sum/2
  Zero-Order Hold/1 -> MATLAB Function/1(valor)
  Transport Delay/1 -> Sum/1
  Integrator3/1 -> MATLAB Function1/2(vel2)  "vel_motor m/s"
  Acel/1 -> Integrator3/1, Integrator2/1, Zero-Order Hold/1, Scope/1
  [run] -> MATLAB Function1/3(run)
  Integrator2/1 -> MATLAB Function1/1(vel1)  "vel_motor m/s"

== system Control_LIM_H9/Modelado completo del motor DLIM/Sensor de Corriente ==
  Corriente UVW : Inport
  Demux : Demux  Outputs=3
  Mux : Mux  Inputs=3
  Scope : Scope
  Sensor corriente U : Subsystem
  Sensor corriente V : Subsystem
  Sensor corriente W : Subsystem
  Corriente Medida : Outport
  wires:
  Corriente UVW/1 -> Scope/1, Demux/1
  Demux/1 -> Sensor corriente U/1(I)
  Demux/2 -> Sensor corriente V/1(I)
  Demux/3 -> Sensor corriente W/1(I)
  Mux/1 -> Corriente Medida/1
  Sensor corriente U/1(valor) -> Mux/1
  Sensor corriente W/1(valor) -> Mux/3
  Sensor corriente V/1(valor) -> Mux/2

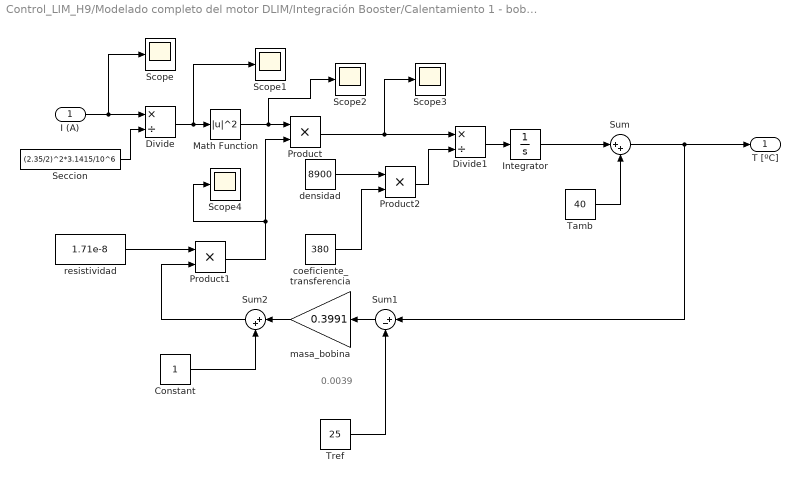
== system Control_LIM_H9/Modelado completo del motor DLIM/Integración Booster/Calentamiento 1 - bobina ==
  note: 0.0039
  I (A) : Inport
  Constant : Constant
  Divide : Product  Inputs=*/
  Divide1 : Product  Inputs=*/
  Integrator : Integrator
  Math Function : Math  Operator=magnitude^2
  Product : Product
  Product1 : Product
  Product2 : Product
  Scope{,1..4} (5 alike) : Scope
      Scope settings: ActiveDisplayYMinimum=-124.99997  ActiveDisplayYMaximum=125  DataLoggingVariableName=ScopeData10
      Scope1 settings: DataLoggingVariableName=ScopeData11
      Scope2 settings: DataLoggingVariableName=ScopeData12
      Scope3 settings: DataLoggingVariableName=ScopeData13
      Scope4 settings: DataLoggingVariableName=ScopeData14
  Seccion : Constant  Value=(2.35/2)^2*3.1415/10^6
  Sum : Sum  Inputs=|++
  Sum1 : Sum  Inputs=|+-
  Sum2 : Sum  Inputs=|++
  Tamb : Constant  Value=40
  Tref : Constant  Value=25
  coeficiente_transferencia : Constant  Value=380
  densidad : Constant  Value=8900
  masa_bobina : Gain  Gain=0.3991
  resistividad : Constant  Value=1.71e-8
  T [ºC] : Outport
  wires:
  I (A)/1 -> Scope/1, Divide/1
  Seccion/1 -> Divide/2
  Divide/1 -> Scope1/1, Math Function/1
  Math Function/1 -> Scope2/1, Product/1
  Product/1 -> Scope3/1, Divide1/1
  Divide1/1 -> Integrator/1
  Integrator/1 -> Sum/1
  Tamb/1 -> Sum/2
  Sum/1 -> Sum1/1, T [ºC]/1
  Sum1/1 -> masa_bobina/1
  Tref/1 -> Sum1/2
  masa_bobina/1 -> Sum2/1
  Constant/1 -> Sum2/2
  resistividad/1 -> Product1/1
  Sum2/1 -> Product1/2
  Product1/1 -> Scope4/1, Product/2
  Product2/1 -> Divide1/2
  densidad/1 -> Product2/1
  coeficiente_transferencia/1 -> Product2/2

== system Control_LIM_H9/Modelado completo del motor DLIM/Integración Booster/From x to fp ==
  In1 : Inport
  Constant : Constant  Value=0.032
  Constant1 : Constant  Value=2
  Divide : Product  Inputs=*/
  Divide1 : Product  Inputs=*/
  Gain : Gain  Gain=2
  Round : Rounding
  Sum : Sum  Inputs=|+-
  Out1 : Outport
  wires:
  In1/1 -> Divide/1
  Constant/1 -> Divide/2
  Divide/1 -> Divide1/1, Sum/1
  Divide1/1 -> Round/1
  Round/1 -> Gain/1
  Constant1/1 -> Divide1/2
  Gain/1 -> Sum/2
  Sum/1 -> Out1/1

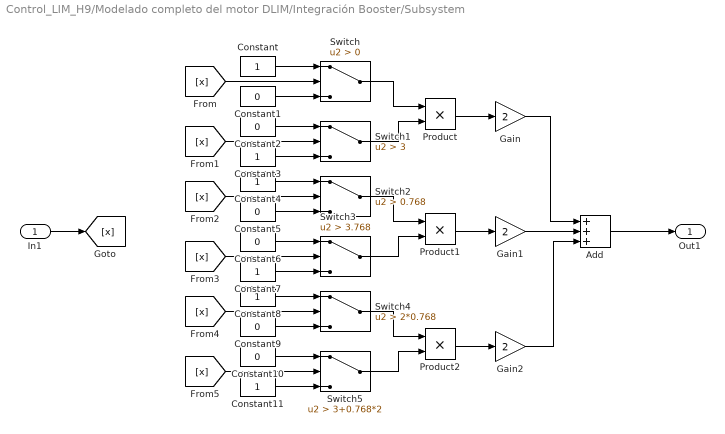
== system Control_LIM_H9/Modelado completo del motor DLIM/Integración Booster/Subsystem ==
  In1 : Inport
  Add : Sum  Inputs=+++
  Constant{,3..4,7..8,11} (6 alike) : Constant
  Constant{1..2,5..6,9..10} (6 alike) : Constant  Value=0
  Gain : Gain  Gain=2
  Gain1 : Gain  Gain=2
  Gain2 : Gain  Gain=2
  Product : Product
  Product1 : Product
  Product2 : Product
  Switch : Switch  Criteria=u2 > Threshold  SaturateOnIntegerOverflow=off  InputSameDT=off
  Switch1 : Switch  Criteria=u2 > Threshold  Threshold=3  SaturateOnIntegerOverflow=off  InputSameDT=off
  Switch2 : Switch  Criteria=u2 > Threshold  Threshold=0.768  SaturateOnIntegerOverflow=off  InputSameDT=off
  Switch3 : Switch  Criteria=u2 > Threshold  Threshold=3.768  SaturateOnIntegerOverflow=off  InputSameDT=off
  Switch4 : Switch  Criteria=u2 > Threshold  Threshold=2*0.768  SaturateOnIntegerOverflow=off  InputSameDT=off
  Switch5 : Switch  Criteria=u2 > Threshold  Threshold=3+0.768*2  SaturateOnIntegerOverflow=off  InputSameDT=off
  Out1 : Outport
  wires:
  In1/1 -> [x]
  Add/1 -> Out1/1
  Product/1 -> Gain/1
  Constant1/1 -> Switch/3
  Switch/1 -> Product/1
  Product2/1 -> Gain2/1
  Gain1/1 -> Add/2
  [x] -> Switch/2
  Constant2/1 -> Switch1/1
  [x] -> Switch1/2
  Constant/1 -> Switch/1
  Switch5/1 -> Product2/2
  Switch1/1 -> Product/2
  Switch3/1 -> Product1/2
  Switch2/1 -> Product1/1
  Constant10/1 -> Switch5/1
  [x] -> Switch5/2
  Constant11/1 -> Switch5/3
  Gain/1 -> Add/1
  Product1/1 -> Gain1/1
  [x] -> Switch3/2
  Gain2/1 -> Add/3
  [x] -> Switch2/2
  Constant8/1 -> Switch4/1
  Constant6/1 -> Switch3/1
  Constant9/1 -> Switch4/3
  Constant3/1 -> Switch1/3
  Constant4/1 -> Switch2/1
  Constant7/1 -> Switch3/3
  Constant5/1 -> Switch2/3
  [x] -> Switch4/2
  Switch4/1 -> Product2/1

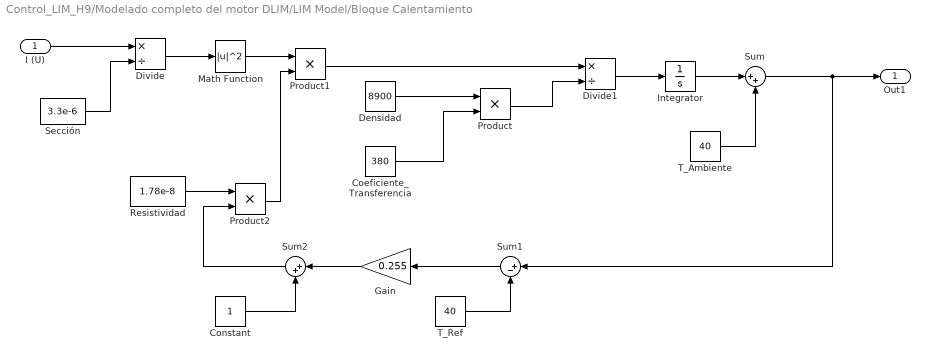
== system Control_LIM_H9/Modelado completo del motor DLIM/LIM Model/Bloque Calentamiento ==
  I (U) : Inport
  Coeficiente_Transferencia : Constant  Value=380
  Constant : Constant
  Densidad : Constant  Value=8900
  Divide : Product  Inputs=*/
  Divide1 : Product  Inputs=*/
  Gain : Gain  Gain=0.255
  Integrator : Integrator
  Math Function : Math  Operator=magnitude^2
  Product : Product
  Product1 : Product
  Product2 : Product
  Resistividad : Constant  Value=1.78e-8
  Sección : Constant  Value=3.3e-6
  Sum : Sum  Inputs=|++
  Sum1 : Sum  Inputs=|+-
  Sum2 : Sum  Inputs=|++
  T_Ambiente : Constant  Value=40
  T_Ref : Constant  Value=40
  Out1 : Outport
  wires:
  I (U)/1 -> Divide/1
  Sección/1 -> Divide/2
  Divide/1 -> Math Function/1
  Densidad/1 -> Product/1
  Coeficiente_Transferencia/1 -> Product/2
  Product/1 -> Divide1/2
  Divide1/1 -> Integrator/1
  Math Function/1 -> Product1/1
  Product1/1 -> Divide1/1
  Resistividad/1 -> Product2/1
  Product2/1 -> Product1/2
  Integrator/1 -> Sum/1
  Sum/1 -> Sum1/1, Out1/1
  T_Ambiente/1 -> Sum/2
  Sum1/1 -> Gain/1
  T_Ref/1 -> Sum1/2
  Gain/1 -> Sum2/1
  Constant/1 -> Sum2/2
  Sum2/1 -> Product2/2

== system Control_LIM_H9/Modelado completo del motor DLIM/LIM Model/Cálculo Deslizamiento ==
  note: v_sincronismo = 2 * pp * f
  Frecuencia : Inport
  Velocidad Km/h : Inport  Port=2
  Constant : Constant  Value=paso_polar
  Gain : Gain  Gain=2*3.6
  MATLAB Function : MATLAB Function  TreatAsAtomicUnit=on
  Product : Product
  Scope : Scope  NumInputPorts=3
      settings: ActiveDisplayYMinimum=-1  ActiveDisplayYMaximum=1  DataLoggingVariableName=ScopeData3
  Deslizamiento : Outport
  wires:
  Frecuencia/1 -> Gain/1
  Velocidad Km/h/1 -> Scope/2, MATLAB Function/2(v_motor)
  MATLAB Function/1(slip) -> Scope/3, Deslizamiento/1
  Constant/1 -> Product/1
  Gain/1 -> Product/2
  Product/1 -> MATLAB Function/1(v_sincronismo), Scope/1

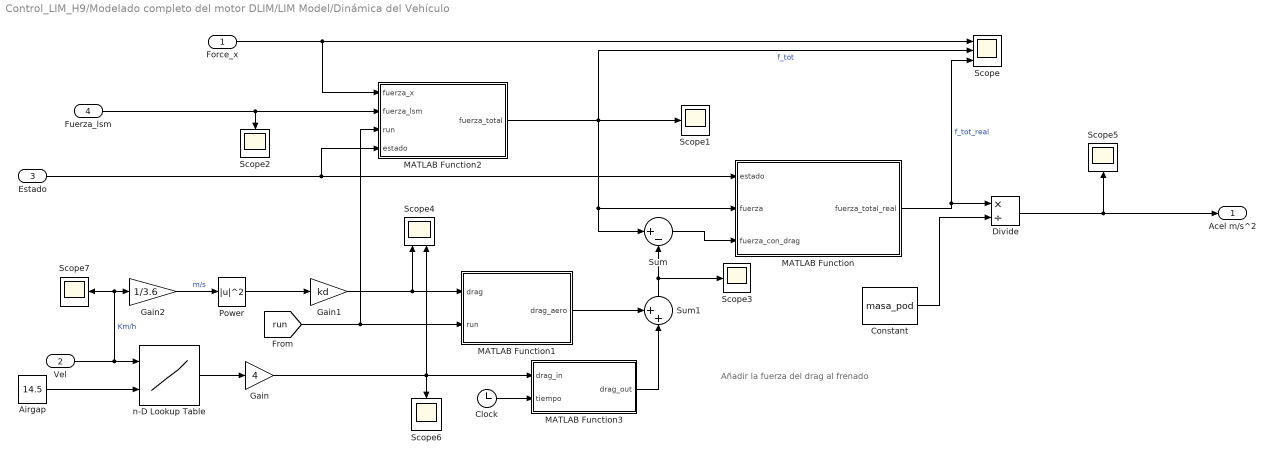
== system Control_LIM_H9/Modelado completo del motor DLIM/LIM Model/Dinámica del Vehículo ==
  note: Añadir la fuerza del drag al frenado
  Force_x : Inport  OutDataTypeStr=double
  Vel : Inport  Port=2
  Estado : Inport  Port=3
  Fuerza_lsm : Inport  Port=4  OutDataTypeStr=double
  Airgap : Constant  Value=14.5
  Clock : Clock
  Constant : Constant  Value=masa_pod
  Divide : Product  Inputs=*/
  Gain : Gain  Gain=4
  Gain1 : Gain  Gain=kd
  Gain2 : Gain  Gain=1/3.6
  MATLAB Function : MATLAB Function  TreatAsAtomicUnit=on
  MATLAB Function1 : MATLAB Function  TreatAsAtomicUnit=on
  MATLAB Function2 : MATLAB Function  TreatAsAtomicUnit=on
  MATLAB Function3 : MATLAB Function  TreatAsAtomicUnit=on
  Power : Math  Operator=magnitude^2
  Scope : Scope  NumInputPorts=3
      settings: ActiveDisplayYMinimum=-4584.62462  ActiveDisplayYMaximum=4049.70577  DataLoggingVariableName=ScopeData22
  Scope{1..3,5..7} (6 alike) : Scope
      Scope1 settings: ActiveDisplayYMinimum=-4356.47364  ActiveDisplayYMaximum=4024.35567
      Scope2 settings: ActiveDisplayYMinimum=-398.32725  ActiveDisplayYMaximum=3584.94528  DataLoggingVariableName=ScopeData2
      Scope3 settings: ActiveDisplayYMinimum=-42.3603  ActiveDisplayYMaximum=381.24267  DataLoggingVariableName=ScopeData7
      Scope5 settings: ActiveDisplayYMinimum=-0.38804  ActiveDisplayYMaximum=0.26651  DataLoggingVariableName=ScopeData13
      Scope6 settings: ActiveDisplayYMinimum=-41.11542  ActiveDisplayYMaximum=370.03797  DataLoggingVariableName=ScopeData14
      Scope7 settings: ActiveDisplayYMinimum=-6.2524  ActiveDisplayYMaximum=56.27152  DataLoggingVariableName=ScopeData15
  Scope4 : Scope  NumInputPorts=2
      settings: ActiveDisplayYMinimum=7.07531  ActiveDisplayYMaximum=33.05629  DataLoggingVariableName=ScopeData11
  Sum : Sum  Inputs=|+-
  Sum1 : Sum  Inputs=++|
  n-D Lookup Table : Lookup_n-D  BreakpointsForDimension1=velocidad_drag  BreakpointsForDimension2=airgap  BreakpointsForDimension3=[5, 7]  Table=fuerza_drag  InternalRulePriority=Speed  RndMeth=Simplest
      settings: InputPortMap=u0,u1
  Acel m/s^2 : Outport
  wires:
  Vel/1 -> Scope7/1, Gain2/1, n-D Lookup Table/1  "Km/h"
  Airgap/1 -> n-D Lookup Table/2
  n-D Lookup Table/1 -> Gain/1
  Force_x/1 -> MATLAB Function2/1(fuerza_x), Scope/1
  Gain/1 -> MATLAB Function3/1(drag_in), Scope4/2, Scope6/1
  Sum/1 -> MATLAB Function/3(fuerza_con_drag)
  Constant/1 -> Divide/2
  Divide/1 -> Scope5/1, Acel m/s^2/1
  MATLAB Function/1(fuerza_total_real) -> Divide/1, Scope/3  "f_tot_real"
  Estado/1 -> MATLAB Function2/4(estado), MATLAB Function/1(estado)
  Power/1 -> Gain1/1
  Gain1/1 -> MATLAB Function1/1(drag), Scope4/1
  [run] -> MATLAB Function1/2(run), MATLAB Function2/3(run)
  Sum1/1 -> Sum/2, Scope3/1
  MATLAB Function1/1(drag_aero) -> Sum1/1
  Fuerza_lsm/1 -> Scope2/1, MATLAB Function2/2(fuerza_lsm)
  MATLAB Function2/1(fuerza_total) -> Scope/2, Scope1/1, Sum/1, MATLAB Function/2(fuerza)  "f_tot"
  Gain2/1 -> Power/1  "m/s"
  MATLAB Function3/1(drag_out) -> Sum1/2
  Clock/1 -> MATLAB Function3/2(tiempo)

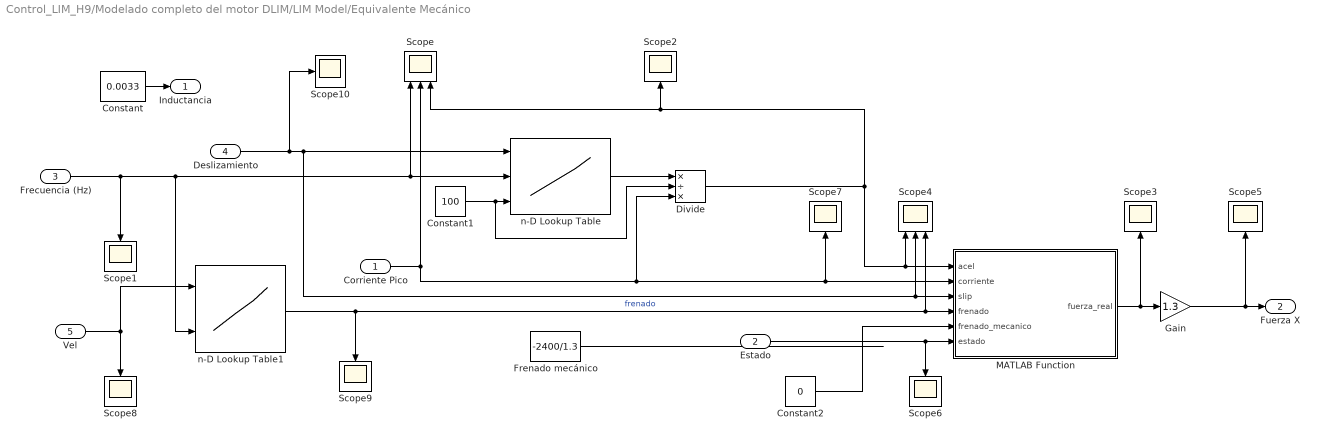
== system Control_LIM_H9/Modelado completo del motor DLIM/LIM Model/Equivalente Mecánico ==
  Corriente Pico : Inport
  Estado : Inport  Port=2
  Frecuencia (Hz) : Inport  Port=3
  Deslizamiento : Inport  Port=4
  Vel : Inport  Port=5
  Constant : Constant  Value=0.0033
  Constant1 : Constant  Value=100
  Constant2 : Constant  Value=0
  Divide : Product  Inputs=*/*
  Frenado mecánico : Constant  Value=-2400/1.3
  Gain : Gain  Gain=1.3  OutDataTypeStr=double
  MATLAB Function : MATLAB Function  TreatAsAtomicUnit=on
  Scope : Scope  NumInputPorts=3
      settings: ActiveDisplayYMinimum=-16.47578  ActiveDisplayYMaximum=118.28206
  Scope{1..3,5..10} (9 alike) : Scope
      Scope1 settings: ActiveDisplayYMinimum=-12.55002  ActiveDisplayYMaximum=82.95022  DataLoggingVariableName=ScopeData3
      Scope2 settings: ActiveDisplayYMinimum=-1159.243  ActiveDisplayYMaximum=10433.187  DataLoggingVariableName=ScopeData10
      Scope3 settings: ActiveDisplayYMinimum=-124.71456  ActiveDisplayYMaximum=1122.43104
      Scope5 settings: ActiveDisplayYMinimum=-4124.50217  ActiveDisplayYMaximum=1936.61247  DataLoggingVariableName=ScopeData2
      Scope6 settings: ActiveDisplayYMinimum=-0.875  ActiveDisplayYMaximum=7.875  DataLoggingVariableName=ScopeData3
      Scope7 settings: ActiveDisplayYMinimum=-13.04512  ActiveDisplayYMaximum=117.40605  DataLoggingVariableName=ScopeData6
      Scope8 settings: ActiveDisplayYMinimum=-6.25133  ActiveDisplayYMaximum=56.26194  DataLoggingVariableName=ScopeData4
      Scope9 settings: ActiveDisplayYMinimum=-2015.88207  ActiveDisplayYMaximum=-177.81443  DataLoggingVariableName=ScopeData5
  Scope4 : Scope  NumInputPorts=3
      settings: ActiveDisplayYMinimum=-3216.44371  ActiveDisplayYMaximum=1883.44948
  n-D Lookup Table : Lookup_n-D  NumberOfTableDimensions=3  BreakpointsForDimension1=slip  BreakpointsForDimension2=frecuencia_acel  BreakpointsForDimension3=corriente  Table=fuerza  InternalRulePriority=Speed  RndMeth=Simplest
      settings: InputPortMap=u0,u1,u2
  n-D Lookup Table1 : Lookup_n-D  BreakpointsForDimension1=vel_motor_freno  BreakpointsForDimension2=frecuencia_freno  BreakpointsForDimension3=[5, 7]  Table=FuerzaX_freno  InternalRulePriority=Speed  RndMeth=Simplest
      settings: InputPortMap=u0,u1
  Inductancia : Outport
  Fuerza X : Outport  Port=2
  wires:
  Divide/1 -> MATLAB Function/1(acel), Scope4/1, Scope2/1, Scope/3
  Corriente Pico/1 -> MATLAB Function/2(corriente), Scope7/1, Divide/3, Scope/2
  Frecuencia (Hz)/1 -> Scope1/1, n-D Lookup Table1/2, n-D Lookup Table/2, Scope/1
  Deslizamiento/1 -> Scope10/1, n-D Lookup Table/1, MATLAB Function/3(slip), Scope4/2
  Vel/1 -> n-D Lookup Table1/1, Scope8/1
  Estado/1 -> Scope6/1, MATLAB Function/6(estado)
  n-D Lookup Table1/1 -> Scope9/1, Scope4/3, MATLAB Function/4(frenado)  "frenado"
  Constant/1 -> Inductancia/1
  Frenado mecánico/1 -> ?
  MATLAB Function/1(fuerza_real) -> Gain/1, Scope3/1
  Gain/1 -> Fuerza X/1, Scope5/1
  Constant1/1 -> Divide/2, n-D Lookup Table/3
  n-D Lookup Table/1 -> Divide/1
  Constant2/1 -> MATLAB Function/5(frenado_mecanico)

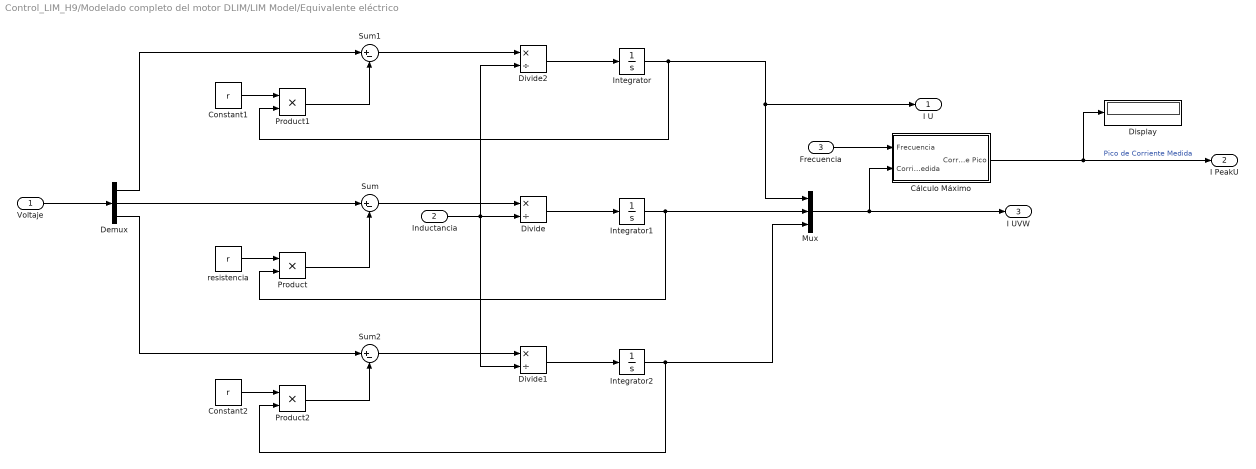
== system Control_LIM_H9/Modelado completo del motor DLIM/LIM Model/Equivalente eléctrico ==
  Voltaje : Inport
  Inductancia : Inport  Port=2
  Frecuencia : Inport  Port=3
  Constant1 : Constant  Value=r
  Constant2 : Constant  Value=r
  Cálculo Máximo : Subsystem
  Demux : Demux  Outputs=3
  Display : Display
  Divide : Product  Inputs=*/
  Divide1 : Product  Inputs=*/
  Divide2 : Product  Inputs=*/
  Integrator : Integrator
  Integrator1 : Integrator
  Integrator2 : Integrator
  Mux : Mux  Inputs=3
  Product : Product
  Product1 : Product
  Product2 : Product
  Sum : Sum  Inputs=|+-
  Sum1 : Sum  Inputs=|+-
  Sum2 : Sum  Inputs=|+-
  resistencia : Constant  Value=r
  I U : Outport
  I PeakU : Outport  Port=2
  I UVW : Outport  Port=3
  wires:
  Voltaje/1 -> Demux/1
  Demux/2 -> Sum/1
  Product/1 -> Sum/2
  resistencia/1 -> Product/1
  Sum/1 -> Divide/1
  Inductancia/1 -> Divide1/2, Divide2/2, Divide/2
  Product1/1 -> Sum1/2
  Sum1/1 -> Divide2/1
  Demux/1 -> Sum1/1
  Constant1/1 -> Product1/1
  Product2/1 -> Sum2/2
  Sum2/1 -> Divide1/1
  Demux/3 -> Sum2/1
  Constant2/1 -> Product2/1
  Divide2/1 -> Integrator/1
  Integrator/1 -> Product1/2, Mux/1, I U/1
  Divide/1 -> Integrator1/1
  Divide1/1 -> Integrator2/1
  Integrator1/1 -> Product/2, Mux/2
  Integrator2/1 -> Product2/2, Mux/3
  Mux/1 -> Cálculo Máximo/2(Corriente Medida), I UVW/1
  Cálculo Máximo/1(Corriente Pico) -> Display/1, I PeakU/1  "Pico de Corriente Medida"
  Frecuencia/1 -> Cálculo Máximo/1(Frecuencia)

== system Control_LIM_H9/Modelado completo del motor DLIM/LIM Model/Velocidad Real ==
  Acel : Inport
  Gain : Gain  Gain=3.6
  Integrator1 : Integrator
  Integrator2 : Integrator  InitialCondition=3/3.6
  MATLAB Function : MATLAB Function  TreatAsAtomicUnit=on
  Scope : Scope  NumInputPorts=2
      settings: ActiveDisplayYMinimum=-0.08727  ActiveDisplayYMaximum=0.01214  DataLoggingVariableName=ScopeData16
  Vel Km/h : Outport
  wires:
  Acel/1 -> Integrator2/1, Integrator1/1, Scope/1  "m/s^2"
  MATLAB Function/1(vel) -> Gain/1  "m/s"
  Gain/1 -> Vel Km/h/1, Scope/2  "Km/h"
  Integrator2/1 -> MATLAB Function/2(vel2)  "vel_motor m/s"
  [run] -> MATLAB Function/3(run)
  Integrator1/1 -> MATLAB Function/1(vel1)  "vel_motor m/s"

== system Control_LIM_H9/Modelado completo del motor DLIM/Sensor de Corriente/Sensor corriente U ==
  I : Inport
  Discretizado Amplitud : MATLAB Function  TreatAsAtomicUnit=on
  MATLAB Function1 : MATLAB Function  TreatAsAtomicUnit=on
  Offset : Constant  Value=0.0001
  Ruido : RandomNumber  Variance=0.000003  Seed=10  SampleTime=0.0002
  Sensor : MATLAB Function  TreatAsAtomicUnit=on
  Sum : Sum  Inputs=|++
  Tiempo Discretizado (s) : ZeroOrderHold  SampleTime=0.0002
  max : Constant  Value=4
  min : Constant
  num_valores : Constant  Value=65535
  valor : Outport
  wires:
  I/1 -> Sensor/1(I)
  Offset/1 -> Sensor/2(Offset)
  Sensor/1(V) -> Sum/1
  Ruido/1 -> Sum/2
  Sum/1 -> Tiempo Discretizado (s)/1
  Tiempo Discretizado (s)/1 -> Discretizado Amplitud/1(valor)
  num_valores/1 -> Discretizado Amplitud/2(num_valores)
  max/1 -> Discretizado Amplitud/3(max)
  min/1 -> Discretizado Amplitud/4(min)
  Discretizado Amplitud/1(valor_discretizado) -> MATLAB Function1/1(V)
  MATLAB Function1/1(I) -> valor/1

== system Control_LIM_H9/Modelado completo del motor DLIM/Sensor de Corriente/Sensor corriente V ==
  I : Inport
  Discretizado Amplitud : MATLAB Function  TreatAsAtomicUnit=on
  MATLAB Function1 : MATLAB Function  TreatAsAtomicUnit=on
  Offset : Constant  Value=0.0001
  Ruido : RandomNumber  Variance=0.000003  Seed=10  SampleTime=0.0002
  Sensor : MATLAB Function  TreatAsAtomicUnit=on
  Sum : Sum  Inputs=|++
  Tiempo Discretizado (s) : ZeroOrderHold  SampleTime=0.0002
  max : Constant  Value=4
  min : Constant
  num_valores : Constant  Value=4096
  valor : Outport
  wires:
  MATLAB Function1/1(I) -> valor/1
  Sensor/1(V) -> Sum/1
  Offset/1 -> Sensor/2(Offset)
  min/1 -> Discretizado Amplitud/4(min)
  Tiempo Discretizado (s)/1 -> Discretizado Amplitud/1(valor)
  Ruido/1 -> Sum/2
  I/1 -> Sensor/1(I)
  Sum/1 -> Tiempo Discretizado (s)/1
  num_valores/1 -> Discretizado Amplitud/2(num_valores)
  Discretizado Amplitud/1(valor_discretizado) -> MATLAB Function1/1(V)
  max/1 -> Discretizado Amplitud/3(max)

== system Control_LIM_H9/Modelado completo del motor DLIM/Sensor de Corriente/Sensor corriente W ==
  I : Inport
  Discretizado Amplitud : MATLAB Function  TreatAsAtomicUnit=on
  MATLAB Function1 : MATLAB Function  TreatAsAtomicUnit=on
  Offset : Constant  Value=0.0001
  Ruido : RandomNumber  Variance=0.000003  Seed=10  SampleTime=0.0002
  Sensor : MATLAB Function  TreatAsAtomicUnit=on
  Sum : Sum  Inputs=|++
  Tiempo Discretizado (s) : ZeroOrderHold  SampleTime=0.0002
  max : Constant  Value=4
  min : Constant
  num_valores : Constant  Value=4096
  valor : Outport
  wires:
  MATLAB Function1/1(I) -> valor/1
  Sensor/1(V) -> Sum/1
  Offset/1 -> Sensor/2(Offset)
  min/1 -> Discretizado Amplitud/4(min)
  Tiempo Discretizado (s)/1 -> Discretizado Amplitud/1(valor)
  Ruido/1 -> Sum/2
  I/1 -> Sensor/1(I)
  Sum/1 -> Tiempo Discretizado (s)/1
  num_valores/1 -> Discretizado Amplitud/2(num_valores)
  Discretizado Amplitud/1(valor_discretizado) -> MATLAB Function1/1(V)
  max/1 -> Discretizado Amplitud/3(max)

== system Control_LIM_H9/Modelado completo del motor DLIM/LIM Model/Equivalente eléctrico/Cálculo Máximo ==
  Frecuencia : Inport
  Corriente Medida : Inport  Port=2
  Clock : Clock
  MATLAB Function : MATLAB Function  TreatAsAtomicUnit=on
  Corriente Pico : Outport
  wires:
  Frecuencia/1 -> MATLAB Function/1(frecuencia)
  MATLAB Function/1(maximo) -> Corriente Pico/1
  Corriente Medida/1 -> MATLAB Function/2(valores)
  Clock/1 -> MATLAB Function/3(tiempo)

== matlab function Control_LIM_H9/Modelado completo del motor DLIM/Sensor de Corriente/Sensor corriente U/MATLAB Function1 ==
  data: V input; I output
function I = fcn(V)

I = (V - 2.5)/0.005;

== matlab function Control_LIM_H9/Modelado completo del motor DLIM/Sensor de Corriente/Sensor corriente V/Discretizado Amplitud ==
  data: valor input; valor_discretizado output; num_valores input; max input; min input
function valor_discretizado = fcn(valor, num_valores, max, min)

if valor > max
    valor_discretizado = max;
    return
end

if valor < min
    valor_discretizado = min;
    return
end


valor_escalon = (max - min)/(num_valores - 1);


i = min;


while (i < max)
    if (i + valor_escalon/2 > valor)
        valor_discretizado = i;
        return
    end

    i = i + valor_escalon;
end


valor_discretizado = max;

end

== matlab function Control_LIM_H9/Modelado completo del motor DLIM/Sensor de Corriente/Sensor corriente V/MATLAB Function1 ==
  data: V input; I output
function I = fcn(V)

I = (V - 2.5)/0.005;

== matlab function Control_LIM_H9/Modelado completo del motor DLIM/Sensor de Corriente/Sensor corriente V/Sensor ==
  data: I input; V output; Offset input
function V = fcn(I, Offset)

Vcc = 5;                                        %Vcc ??                             La corriente va hasta máximo 5V

if (I > 300)
    I = 300;
end

if (I < -300)
    I = -300;
end


V_ref = Vcc / 2;

V = V_ref + 0.005 * I;

V = V + Offset;                 % Por?


end

== matlab function Control_LIM_H9/Modelado completo del motor DLIM/Sensor de Corriente/Sensor corriente W/Discretizado Amplitud ==
  data: valor input; valor_discretizado output; num_valores input; max input; min input
function valor_discretizado = fcn(valor, num_valores, max, min)

if valor > max
    valor_discretizado = max;
    return
end

if valor < min
    valor_discretizado = min;
    return
end


valor_escalon = (max - min)/(num_valores - 1);


i = min;


while (i < max)
    if (i + valor_escalon/2 > valor)
        valor_discretizado = i;
        return
    end

    i = i + valor_escalon;
end


valor_discretizado = max;

end

== matlab function Control_LIM_H9/Modelado completo del motor DLIM/Sensor de Corriente/Sensor corriente W/MATLAB Function1 ==
  data: V input; I output
function I = fcn(V)

I = (V - 2.5)/0.005;

== matlab function Control_LIM_H9/Modelado completo del motor DLIM/Sensor de Corriente/Sensor corriente W/Sensor ==
  data: I input; V output; Offset input
function V = fcn(I, Offset)

Vcc = 5;                                        %Vcc ??                             La corriente va hasta máximo 5V

if (I > 300)
    I = 300;
end

if (I < -300)
    I = -300;
end


V_ref = Vcc / 2;

V = V_ref + 0.005 * I;

V = V + Offset;                 % Por?


end

== matlab function Control_LIM_H9/Modelado completo del motor DLIM/LIM Model/Cálculo Deslizamiento/MATLAB Function ==
  data: v_sincronismo input; slip output; v_motor input
function slip = fcn(v_sincronismo, v_motor)

slip = (v_sincronismo - v_motor) / v_sincronismo;

== matlab function Control_LIM_H9/Control de Velocidad/MATLAB Function ==
  data: i input; i_ref output; estado input; reset output
function [i_ref, reset] = fcn(i, estado)

i_ref=0;

if estado==5 || estado==0 || estado == 7
    i_ref=0;
    reset=1;
else
    reset=0;
    if (estado==2 || estado == 4 || estado == 1 || estado == 6) && i>0
        i_ref=i;
    end
end

== matlab function Control_LIM_H9/Modelado completo del motor DLIM/LIM Model/Equivalente Mecánico/MATLAB Function ==
  data: acel input; corriente input; slip input; frenado input; frenado_mecanico input; estado input; fuerza_real output
function fuerza_real = fcn(acel, corriente, slip, frenado, frenado_mecanico, estado)

if estado == 5 || estado == 6
    fuerza = frenado;
elseif estado == 7
    fuerza = frenado_mecanico;
else
    fuerza = acel;          
end


if slip == 0 || (estado ~= 7 && (estado ~= 5 && (corriente < 6 && corriente > -6))) || estado == 0   %  slip == 0 || (estado ~= 7 && (corriente < 6 && corriente > -6)) || estado == 0
    fuerza_real = 0;
else
    fuerza_real = fuerza;
end
